simulink model "OL_MMC_dqn_GIThub"  (R2024a)
settings: Solver=FixedStepDiscrete  StartTime=0.0  StopTime=2.5  RelTol=1e-3
values from neighbouring files (symbols this model uses):
  f1 = fg    [mmc_dp_hss_vs_simulink_dqn.m]
  fg = 50    [OL_TD_DP_HSS_dqn.m]
  fh = 150    [mmc_dp_hss_vs_simulink_dqn.m]
  flag_hAC = 0    [mmc_dp_hss_vs_simulink_dqn.m]
  il0 = zSS0(4:6)    [mmc_dp_hss_vs_simulink_dqn.m]
  iu0 = zSS0(1:3)    [mmc_dp_hss_vs_simulink_dqn.m]
  kdcL = 1    [mmc_dp_hss_vs_simulink_dqn.m]
  Low_arm_gain = Nsm/Csm    [mmc_dp_hss_vs_simulink_dqn.m]
  m = 0.85    [OL_TD_DP_HSS_dqn.m]
  mStepRel = 0    [mmc_dp_hss_vs_simulink_dqn.m]
  N = 1    [mmc_dp_hss_vs_simulink_dqn.m]
  p = [p, i]    [OL_TD_DP_HSS_dqn.m]
  phMod = pi/2 + delta + [0, -2*pi/3, 2*pi/3]    [mmc_dp_hss_vs_simulink_dqn.m]
  SOL =     [SOL.mat]
  su = -1    [mmc_dp_hss_vs_simulink_dqn.m]
  su_f = -1    [mmc_dp_hss_vs_simulink_dqn.m]
  T_dc = 0.66    [mmc_dp_hss_vs_simulink_dqn.m]
  t_entranceHF = 0.65    [mmc_dp_hss_vs_simulink_dqn.m]
  Ts_log = Tp/M    [mmc_dp_hss_vs_simulink_dqn.m]
  tStep = Tss    (= 0.6)    [mmc_dp_hss_vs_simulink_dqn.m]
  vC0_sl = zSS0(7:12)    [mmc_dp_hss_vs_simulink_dqn.m]
  Vg_sim = complex([[0 1i*Vpeak; 0 0; 0 0], zeros(3, N+2)])    [mmc_dp_hss_vs_simulink_dqn.m]
  Vpeak = Vac_pk    [mmc_dp_hss_vs_simulink_dqn.m]
undefined symbols (not defined in the file or in its folder): DiscIntNeverNeededParam, S, SY3
libraries: DQsym_Lib x19, spsControlledVoltageSourceLib x11, spsSeriesRLCBranchLib x10, spsCurrentMeasurementLib x6, spsGroundLib x4, spsThreePhaseVIMeasurementLib x1, spspowerguiLib x1
settings Model: Creator=salsarayreh  LastModifiedBy=salsarayreh
settings DataIOCC: SaveFinalState=on  SaveOperatingPoint=on  SaveFormat=Array  SaveState=on  ReturnWorkspaceOutputs=off

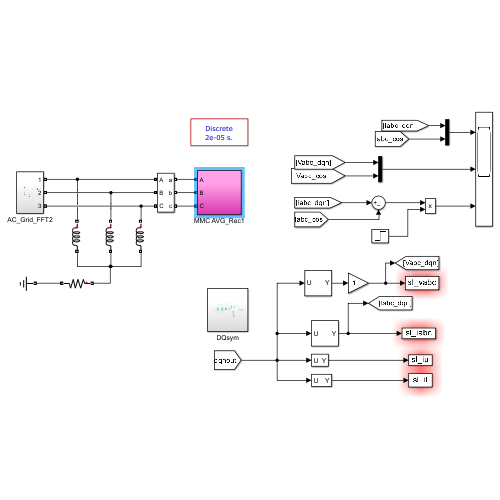
[thumbnail: Simulink's stored preview of the top-level diagram]
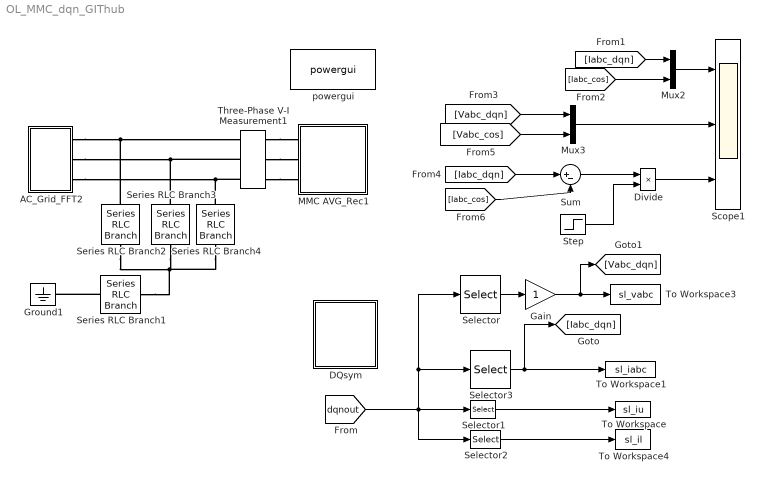
== system OL_MMC_dqn_GIThub ==
  AC_Grid_FFT2 : Subsystem
  DQsym : Subsystem
  Divide : Product  Inputs=**
  Gain : Gain
  Ground1 : spsGroundLib/Ground  LConnTagsString=a
  MMC AVG_Rec1 : Subsystem
  Mux2 : Mux  Inputs=2
  Mux3 : Mux  Inputs=2
  Scope1 : Scope  NumInputPorts=3
  Selector : Selector  InputPortWidth=12  IndexOptions=Index vector (dialog)  Indices=[1:3]  OutputSizes=1
  Selector1 : Selector  InputPortWidth=12  IndexOptions=Index vector (dialog)  Indices=[4:6]  OutputSizes=1
  Selector2 : Selector  InputPortWidth=12  IndexOptions=Index vector (dialog)  Indices=[7:9]  OutputSizes=1
  Selector3 : Selector  InputPortWidth=12  IndexOptions=Index vector (dialog)  Indices=[10:12]  OutputSizes=1
  Series RLC Branch1 : spsSeriesRLCBranchLib/Series RLC Branch  LConnTagsString=__new0  RConnTagsString=__new0  BranchType=R  Resistance=10  Inductance=1e-3  SetiL0=off  InitialCurrent=0  Capacitance=1e-6  Setx0=off  InitialVoltage=0  Measurements=None
  Series RLC Branch2 : spsSeriesRLCBranchLib/Series RLC Branch  LConnTagsString=__new0  RConnTagsString=__new0  BranchType=L  Resistance=10  Inductance=5  SetiL0=off  InitialCurrent=0  Capacitance=1e-6  Setx0=off  InitialVoltage=0  Measurements=None
  Series RLC Branch3 : spsSeriesRLCBranchLib/Series RLC Branch  LConnTagsString=__new0  RConnTagsString=__new0  BranchType=L  Resistance=10  Inductance=5  SetiL0=off  InitialCurrent=0  Capacitance=1e-6  Setx0=off  InitialVoltage=0  Measurements=None
  Series RLC Branch4 : spsSeriesRLCBranchLib/Series RLC Branch  LConnTagsString=__new0  RConnTagsString=__new0  BranchType=L  Resistance=10  Inductance=5  SetiL0=off  InitialCurrent=0  Capacitance=1e-6  Setx0=off  InitialVoltage=0  Measurements=None
  Step : Step  Time=0.5  SampleTime=0
  Sum : Sum  Inputs=|+-
  Three-Phase V-I Measurement1 : spsThreePhaseVIMeasurementLib/Three-Phase V-I Measurement  VoltageMeasurement=phase-to-ground  SetLabelV=on  LabelV=Vabc_cos  Vpu=off  VpuLL=off  CurrentMeasurement=yes  SetLabelI=on  LabelI=Iabc_cos  Ipu=off  Pbase=100e6  Vbase=500e3  OutputType=Complex  PhasorSimulation=off  PSBequivalent=0
  To Workspace : ToWorkspace  VariableName=sl_iu  SaveFormat=Timeseries  SampleTime=Ts_log
  To Workspace1 : ToWorkspace  VariableName=sl_iabc  SaveFormat=Timeseries  SampleTime=Ts_log
  To Workspace3 : ToWorkspace  VariableName=sl_vabc  SaveFormat=Timeseries  SampleTime=Ts_log
  To Workspace4 : ToWorkspace  VariableName=sl_il  SaveFormat=Timeseries  SampleTime=Ts_log
  powergui : spspowerguiLib/powergui  Priority=1  SimulationMode=Discrete  SampleTime=2e-5  frequency=60  Iterations=50  frequencyindice=0  Pbase=100e6  ErrMax=1e-4  UnitsV=kV  UnitsW=MW  buscounter=0  FunctionMessages=off  echomessages=off  EnableUseOfTLC=off  CurrentSourceSwitches=off  DisableSnubberDevices=off  DisableRonSwitches=off  DisableVfSwitches=off  DisplayEquations=off  AutomaticDiscreteSolvers=off  SolverType=Tustin/Backward Euler (TBE)  Interpol=off  ExternalGateDelay=off  methode=off  Ts=10  x0status=blocks  SPID=off  SwTol=0  HookPort=off  NonlinearTolerance=1e-4  nMaxIteration=100  ContinueOnMaxIteration=off  RestoreLinks=warning  ResistiveCurrentMeasurement=off  Frange=[0:2:500]  Ylog=off  Xlog=on  ShowGrid=off  save=off  variable=ZData  structure=VIprim  ZoomFFT=on  StartTime=0.15  cycles=2  DisplayStyle=1  fundamental=50  FreqAxis=on  MaxFrequency=1000  frequencyindicesteady=1  RmsSteady=1  display=off
  wires:
  Selector3/1 -> To Workspace1/1, [Iabc_dqn]
  Selector/1 -> Gain/1
  Gain/1 -> [Vabc_dqn], To Workspace3/1
  [dqnout] -> Selector/1, Selector3/1, Selector2/1, Selector1/1
  [Vabc_cos] -> Mux3/2
  [Iabc_cos] -> Mux2/2
  Mux2/1 -> Scope1/1
  Mux3/1 -> Scope1/2
  Selector2/1 -> To Workspace4/1
  Selector1/1 -> To Workspace/1
  Divide/1 -> Scope1/3
  Sum/1 -> Divide/1
  Step/1 -> Divide/2
  [Iabc_dqn] -> Mux2/1
  [Vabc_dqn] -> Mux3/1
  [Iabc_dqn] -> Sum/1
  [Iabc_cos] -> Sum/2
  connections:
  Series RLC Branch1/LConn1 -- Series RLC Branch2/RConn1 -- Series RLC Branch4/RConn1 -- Series RLC Branch3/RConn1
  Three-Phase V-I Measurement1/LConn2 -- Series RLC Branch3/LConn1 -- AC_Grid_FFT2/LConn2
  Three-Phase V-I Measurement1/LConn3 -- AC_Grid_FFT2/LConn3 -- Series RLC Branch4/LConn1
  AC_Grid_FFT2/LConn1 -- Three-Phase V-I Measurement1/LConn1 -- Series RLC Branch2/LConn1
  Series RLC Branch1/RConn1 -- Ground1/LConn1
  Three-Phase V-I Measurement1/RConn2 -- MMC AVG_Rec1/LConn2
  Three-Phase V-I Measurement1/RConn3 -- MMC AVG_Rec1/LConn3
  Three-Phase V-I Measurement1/RConn1 -- MMC AVG_Rec1/LConn1

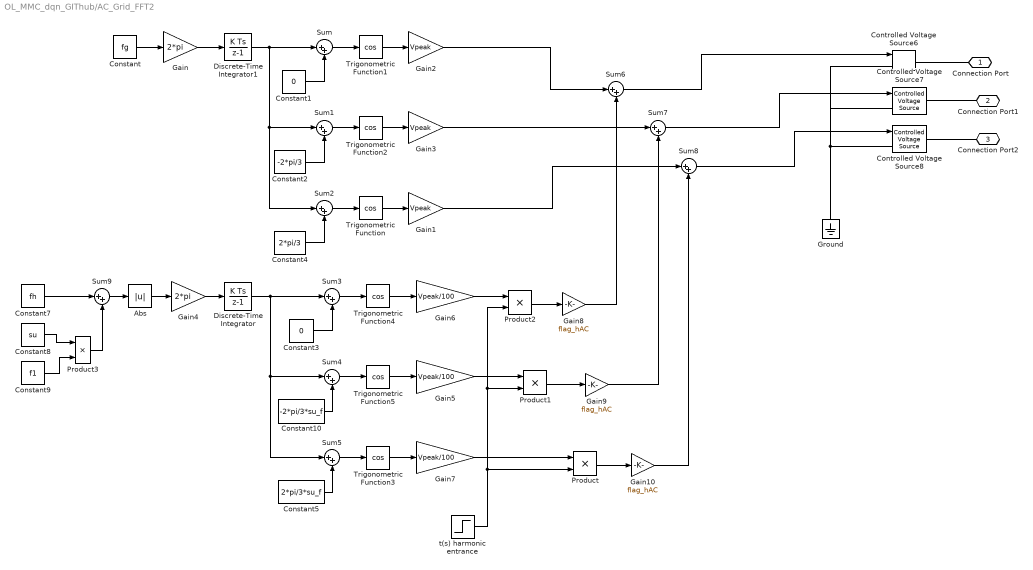
== system OL_MMC_dqn_GIThub/AC_Grid_FFT2 ==
  Abs : Abs  SaturateOnIntegerOverflow=off
  Constant : Constant  Value=fg
  Constant1 : Constant  Value=0
  Constant10 : Constant  Value=-2*pi/3*su_f
  Constant2 : Constant  Value=-2*pi/3
  Constant3 : Constant  Value=0
  Constant4 : Constant  Value=2*pi/3
  Constant5 : Constant  Value=2*pi/3*su_f
  Constant7 : Constant  Value=fh
  Constant8 : Constant  Value=su
  Constant9 : Constant  Value=f1
  Controlled Voltage Source6 : spsControlledVoltageSourceLib/Controlled Voltage Source  Initialize=on  Source_Type=AC  Amplitude=0  Phase=0  Frequency=0  Measurements=None
  Controlled Voltage Source7 : spsControlledVoltageSourceLib/Controlled Voltage Source  Initialize=on  Source_Type=AC  Amplitude=0  Phase=0  Frequency=0  Measurements=None
  Controlled Voltage Source8 : spsControlledVoltageSourceLib/Controlled Voltage Source  Initialize=on  Source_Type=AC  Amplitude=0  Phase=0  Frequency=0  Measurements=None
  Discrete-Time Integrator : DiscreteIntegrator  SampleTime=-1  ICPrevOutput=DiscIntNeverNeededParam  ICPrevScaledInput=DiscIntNeverNeededParam
  Discrete-Time Integrator1 : DiscreteIntegrator  SampleTime=-1  ICPrevOutput=DiscIntNeverNeededParam  ICPrevScaledInput=DiscIntNeverNeededParam
  Gain : Gain  Gain=2*pi
  Gain1 : Gain  Gain=Vpeak
  Gain10 : Gain  Gain=flag_hAC
  Gain2 : Gain  Gain=Vpeak
  Gain3 : Gain  Gain=Vpeak
  Gain4 : Gain  Gain=2*pi
  Gain5 : Gain  Gain=Vpeak/100
  Gain6 : Gain  Gain=Vpeak/100
  Gain7 : Gain  Gain=Vpeak/100
  Gain8 : Gain  Gain=flag_hAC
  Gain9 : Gain  Gain=flag_hAC
  Ground : spsGroundLib/Ground  LConnTagsString=a
  Product{,1..3} (4 alike) : Product
  Sum{,1..9} (10 alike) : Sum  Inputs=|++
  Trigonometric Function{,1..5} (6 alike) : Trigonometry  Operator=cos
  t(s) harmonic entrance : Step  Time=t_entranceHF  SampleTime=0
  Connection Port : PMIOPort  Side=Left
  Connection Port1 : PMIOPort  Port=2  Side=Left
  Connection Port2 : PMIOPort  Port=3  Side=Left
  wires:
  Constant9/1 -> Product3/2
  Product3/1 -> Sum9/2
  Constant8/1 -> Product3/1
  Sum9/1 -> Abs/1
  Constant7/1 -> Sum9/1
  Abs/1 -> Gain4/1
  t(s) harmonic entrance/1 -> Product1/2, Product2/2, Product/2
  Gain5/1 -> Product1/1
  Gain6/1 -> Product2/1
  Constant5/1 -> Sum5/2
  Trigonometric Function1/1 -> Gain2/1
  Constant3/1 -> Sum3/2
  Sum4/1 -> Trigonometric Function5/1
  Discrete-Time Integrator1/1 -> Sum/1, Sum1/1, Sum2/1
  Constant2/1 -> Sum1/2
  Constant10/1 -> Sum4/2
  Constant4/1 -> Sum2/2
  Sum2/1 -> Trigonometric Function/1
  Trigonometric Function3/1 -> Gain7/1
  Sum/1 -> Trigonometric Function1/1
  Trigonometric Function2/1 -> Gain3/1
  Gain/1 -> Discrete-Time Integrator1/1
  Sum5/1 -> Trigonometric Function3/1
  Constant/1 -> Gain/1
  Trigonometric Function/1 -> Gain1/1
  Sum3/1 -> Trigonometric Function4/1
  Gain4/1 -> Discrete-Time Integrator/1
  Gain3/1 -> Sum7/1
  Gain2/1 -> Sum6/1
  Trigonometric Function5/1 -> Gain5/1
  Trigonometric Function4/1 -> Gain6/1
  Constant1/1 -> Sum/2
  Gain7/1 -> Product/1
  Gain1/1 -> Sum8/1
  Sum1/1 -> Trigonometric Function2/1
  Discrete-Time Integrator/1 -> Sum5/1, Sum4/1, Sum3/1
  Product2/1 -> Gain8/1
  Product1/1 -> Gain9/1
  Product/1 -> Gain10/1
  Sum6/1 -> Controlled Voltage Source6/1
  Sum8/1 -> Controlled Voltage Source8/1
  Sum7/1 -> Controlled Voltage Source7/1
  Gain8/1 -> Sum6/2
  Gain9/1 -> Sum7/2
  Gain10/1 -> Sum8/2
  connections:
  Ground/LConn1 -- Controlled Voltage Source6/LConn1 -- Controlled Voltage Source7/LConn1 -- Controlled Voltage Source8/LConn1
  Connection Port/RConn1 -- Controlled Voltage Source6/RConn1
  Connection Port1/RConn1 -- Controlled Voltage Source7/RConn1
  Connection Port2/RConn1 -- Controlled Voltage Source8/RConn1

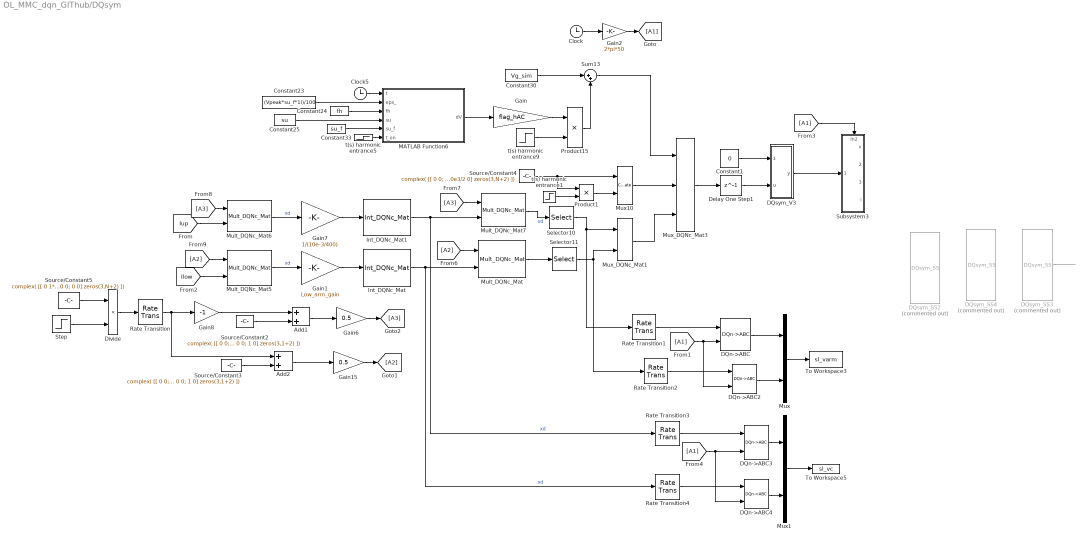
== system OL_MMC_dqn_GIThub/DQsym ==
  Add1 : Sum
  Add2 : Sum
  Clock : Clock
  Clock5 : Clock
  Constant1 : Constant  Value=0
  Constant23 : Constant  Value=(Vpeak*su_f*1i)/100
  Constant24 : Constant  Value=fh
  Constant25 : Constant  Value=su
  Constant30 : Constant  Value=Vg_sim
  Constant33 : Constant  Value=su_f
  DQn->ABC{,2..4} (4 alike) : DQsym_Lib/DQn->ABC  N=4
      settings: SourceProductName=DQsym Library
  DQsym_SS2 : DQsym_Lib/DQsym_SS  Commented=on  Ad=SOL.A  Bd=SOL.B  Cd=SOL.C  Dd=SOL.D  f=fg  swOnRes=0  swOffRes=0  swType=0  Ts=2e-5  nrSWvec=0  xo=SOL.x0
      settings: SourceProductName=DQsym Library
  DQsym_SS3 : DQsym_Lib/DQsym_SS  Commented=on  Ad=Ad1  Bd=Bd1  Cd=Cd1  Dd=Dd1  f=Fnom  swOnRes=1e-3*ones(1,6)  swOffRes=1e6*ones(1,6)  swType=zeros(1,6)  Ts=2e-5  nrSWvec=0  xo=zeros(6,1)
      settings: SourceProductName=DQsym Library
  DQsym_SS4 : DQsym_Lib/DQsym_SS  Commented=on  Ad=ds.A  Bd=ds.B  Cd=ds.C  Dd=ds.D  f=Fnom  swOnRes=1e-3*ones(1,6)  swOffRes=1e6*ones(1,6)  swType=zeros(1,6)  Ts=2e-5  nrSWvec=0  xo=zeros(6,1)
      settings: SourceProductName=DQsym Library
  DQsym_V3 : MATLAB Function  AncestorBlock=DQsym_Lib/DQsym_V3  TreatAsAtomicUnit=on  mask{Ad=SOL.A, Bd=SOL.B, Cd=SOL.C, Dd=SOL.D, f=50, swOnRes=0, swOffRes=0, swType=0, Ts=2e-5, nrSWvec=0, xo=zeros(9,1)}
      mask prompts: Ad "A"; Bd "B"; Cd "C"; Dd "D"; f "frequency"; swOnRes "Switch on resistance:"; swOffRes "Switch off resistance:"; swType "Switch type:"; Ts "Time step (s):"; nrSWvec "Number of switches:"; xo "Initial conditions"
  Delay One Step1 : Delay  DelayLength=1  SampleTime=2e-5
  Divide : Product  Inputs=**
  Gain : Gain  Gain=flag_hAC
  Gain1 : Gain  Gain=Low_arm_gain
  Gain15 : Gain  Gain=0.5
  Gain2 : Gain  Gain=2*pi*50
  Gain6 : Gain  Gain=0.5
  Gain7 : Gain  Gain=1/(10e-3/400)
  Gain8 : Gain  Gain=-1
  Int_DQNc_Mat : DQsym_Lib/Int_DQNc_Mat  N=N+7  dt=Ts_dqn  w=2*pi*fg  InitInt=[vC0_sl(4) ;vC0_sl(5);vC0_sl(6)]  swFeed=off  R=eye(3)  iL=eye(3)
      settings: SourceProductName=DQsym Library
  Int_DQNc_Mat1 : DQsym_Lib/Int_DQNc_Mat  N=N+7  dt=Ts_dqn  w=2*pi*fg  InitInt=[vC0_sl(1) ;vC0_sl(2);vC0_sl(3)]  swFeed=off  R=eye(3)  iL=eye(3)
      settings: SourceProductName=DQsym Library
  MATLAB Function6 : MATLAB Function  TreatAsAtomicUnit=on
  Mult_DQNc_Mat : DQsym_Lib/Mult_DQNc_Mat  N=N+9  HrmDbl=on
      settings: SourceProductName=DQsym Library
  Mult_DQNc_Mat5 : DQsym_Lib/Mult_DQNc_Mat  N=N+3  HrmDbl=on
      settings: SourceProductName=DQsym Library
  Mult_DQNc_Mat6 : DQsym_Lib/Mult_DQNc_Mat  N=N+3  HrmDbl=on
      settings: SourceProductName=DQsym Library
  Mult_DQNc_Mat7 : DQsym_Lib/Mult_DQNc_Mat  N=N+9  HrmDbl=on
      settings: SourceProductName=DQsym Library
  Mux : Mux  Inputs=2
  Mux1 : Mux  Inputs=2
  Mux10 : Concatenate  Mode=Multidimensional array
  Mux_DQNc_Mat1 : DQsym_Lib/Mux_DQNc_Mat  nrInp=2
      settings: SourceProductName=DQsym Library
  Mux_DQNc_Mat3 : DQsym_Lib/Mux_DQNc_Mat  nrInp=3
      settings: SourceProductName=DQsym Library
  Product1 : Product
  Product15 : Product
  Rate Transition : RateTransition  OutPortSampleTime=4e-5
  Rate Transition{1..4} (4 alike) : RateTransition  OutPortSampleTime=2e-5
  Selector10 : Selector  NumberOfDimensions=2  InputPortWidth=size(SY3.C,1)  IndexOptions=Select all,Index vector (dialog)  Indices=4:6,1:N+4  OutputSizes=1,1
  Selector11 : Selector  NumberOfDimensions=2  InputPortWidth=size(SY3.C,1)  IndexOptions=Select all,Index vector (dialog)  Indices=4:6,1:N+4  OutputSizes=1,1
  Source/Constant2 : Constant  Value=complex( [[ 0 0; 0 0; 1 0] zeros(3,1+2) ])
  Source/Constant3 : Constant  Value=complex( [[ 0 0; 0 0; 1 0] zeros(3,1+2) ])
  Source/Constant4 : Constant  Value=complex( [[ 0 0; 0 0; 640e3/2 0] zeros(3,N+2) ])
  Source/Constant5 : Constant  Value=complex( [[ 0 1*exp(1i*1.5359); 0 0; 0 0] zeros(3,N+2) ])
  Step : Step  Time=tStep  Before=m  After=m*(1+mStepRel)  SampleTime=0
  Subsystem3 : Subsystem
      settings: PortSchema="{\"entries\":[{\"content\":{\"sides\":[{\"content\":{\"connectorIds\":[\"In1\"]},\"type\":\"ConnectorPlacement.EquallySpacedRectSide\",\"uuid\":\"3bb77d8f-1aaa-4265-9b68-ea1550baad0f\"},{\"content\":{\"connectorIds\":[\"Out1\",\"Out2\",\"Out3\",\"Out4\"],\"side\":\"RIGHT\"},\"type\":\"ConnectorPlacement.EquallySpacedRectSide\",\"uuid\":\"cf9e0e6c-58d6-47ae-94f0-731f989c2c33\"},{\"content\":{\"connectorIds\":[\"In2\"],\"side\":\"TOP\"},\"type\":\"ConnectorPlacement.EquallySpacedRectSide\",\"uuid\":\"a148aa31-b036-466e-b1e9-6b0bda301938\"}]},\"type\":\"ConnectorPlacement.EquallySpacedConnector\",\"uuid\":\"1e5021a9-33df-40ee-a00e-8c2f12721673\"}],\"packageUris\":[\"http://schema.mathworks.com/mf0/Connector/R2020b\"],\"version\":\"1.0\"}"
  Sum13 : Sum  Inputs=|++
  To Workspace3 : ToWorkspace  VariableName=sl_varm  SaveFormat=Timeseries  SampleTime=Ts_log
  To Workspace5 : ToWorkspace  VariableName=sl_vc  SaveFormat=Timeseries  SampleTime=Ts_log
  t(s) harmonic entrance1 : Step  Time=T_dc  Before=1  After=kdcL  SampleTime=0
  t(s) harmonic entrance5 : Step  Time=t_entranceHF  SampleTime=0
  t(s) harmonic entrance9 : Step  Time=t_entranceHF  SampleTime=0
  wires:
  Int_DQNc_Mat1/1 -> Mult_DQNc_Mat7/2, Rate Transition3/1  "xd"
  [A3] -> Mult_DQNc_Mat7/1
  Int_DQNc_Mat/1 -> Mult_DQNc_Mat/2, Rate Transition4/1  "xd"
  Mult_DQNc_Mat5/1 -> Gain1/1  "xd"
  Constant1/1 -> DQsym_V3/1(brkVec)
  [A3] -> Mult_DQNc_Mat6/1
  [Ilow] -> Mult_DQNc_Mat5/2
  Delay One Step1/1 -> DQsym_V3/2(u)
  Selector10/1 -> Mux_DQNc_Mat1/1, Rate Transition1/1
  DQsym_SS3/1 -> ?
  [A2] -> Mult_DQNc_Mat5/1
  [A2] -> Mult_DQNc_Mat/1
  [A1] -> Subsystem3/2(In2)
  Mult_DQNc_Mat7/1 -> Selector10/1  "xd"
  Sum13/1 -> Mux_DQNc_Mat3/1
  ? -> DQsym_SS3/1
  Gain7/1 -> Int_DQNc_Mat1/1
  Selector11/1 -> Mux_DQNc_Mat1/2, Rate Transition2/1
  ? -> DQsym_SS3/2
  Mux_DQNc_Mat3/1 -> Delay One Step1/1
  [Iup] -> Mult_DQNc_Mat6/2
  DQsym_V3/1(y) -> Subsystem3/1(In1)
  Mult_DQNc_Mat6/1 -> Gain7/1  "xd"
  Gain1/1 -> Int_DQNc_Mat/1
  Mult_DQNc_Mat/1 -> Selector11/1
  Mux_DQNc_Mat1/1 -> Mux_DQNc_Mat3/3
  Gain2/1 -> [A1]
  [A1] -> DQn->ABC2/2, DQn->ABC/2
  Clock/1 -> Gain2/1
  Add1/1 -> Gain6/1
  Gain15/1 -> [A2]
  Gain6/1 -> [A3]
  Divide/1 -> Rate Transition/1
  Add2/1 -> Gain15/1
  Source/Constant3/1 -> Add2/2
  Gain8/1 -> Add1/1
  Source/Constant2/1 -> Add1/2
  Step/1 -> Divide/2
  Source/Constant5/1 -> Divide/1
  Mux10/1 -> Mux_DQNc_Mat3/2
  Source/Constant4/1 -> Mux10/1, Product1/1
  DQn->ABC/1 -> Mux/1
  DQn->ABC2/1 -> Mux/2
  Mux/1 -> To Workspace3/1
  Rate Transition/1 -> Add2/1, Gain8/1
  Rate Transition1/1 -> DQn->ABC/1
  Rate Transition2/1 -> DQn->ABC2/1
  Rate Transition4/1 -> DQn->ABC4/1
  Rate Transition3/1 -> DQn->ABC3/1
  Mux1/1 -> To Workspace5/1
  DQn->ABC4/1 -> Mux1/2
  DQn->ABC3/1 -> Mux1/1
  [A1] -> DQn->ABC3/2, DQn->ABC4/2
  Clock5/1 -> MATLAB Function6/1(t)
  Constant33/1 -> MATLAB Function6/5(su_f)
  t(s) harmonic entrance5/1 -> MATLAB Function6/6(t_on)
  Constant23/1 -> MATLAB Function6/2(eps_)
  Constant25/1 -> MATLAB Function6/4(su)
  t(s) harmonic entrance9/1 -> Product15/2
  Constant24/1 -> MATLAB Function6/3(fh)
  Product15/1 -> Sum13/2
  MATLAB Function6/1(dV) -> Gain/1
  Constant30/1 -> Sum13/1
  Gain/1 -> Product15/1
  t(s) harmonic entrance1/1 -> Product1/2
  Product1/1 -> Mux10/2

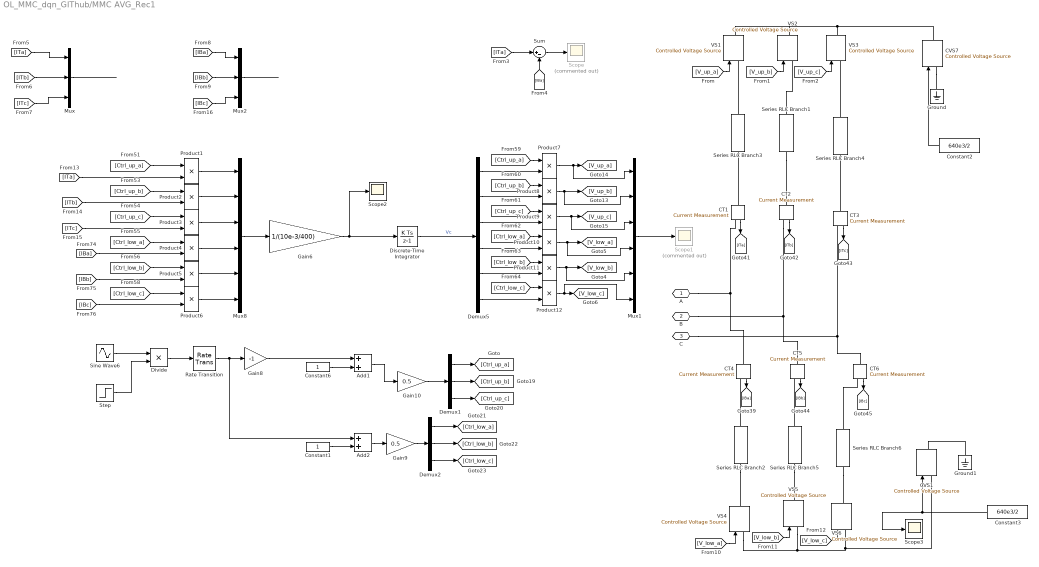
== system OL_MMC_dqn_GIThub/MMC AVG_Rec1 ==
  Add1 : Sum
  Add2 : Sum
  CT{1..6} (6 alike) : spsCurrentMeasurementLib/Current Measurement  PhasorSimulation=off  OutputType=Complex  PSBequivalent=0
  CVS1 : spsControlledVoltageSourceLib/Controlled Voltage Source  Initialize=off  Source_Type=AC  Amplitude=0  Phase=0  Frequency=0  Measurements=None
  CVS7 : spsControlledVoltageSourceLib/Controlled Voltage Source  Initialize=off  Source_Type=AC  Amplitude=0  Phase=0  Frequency=0  Measurements=None
  Constant1 : Constant
  Constant2 : Constant  Value=640e3/2  SampleTime=2e-5
  Constant3 : Constant  Value=640e3/2  SampleTime=2e-5
  Constant6 : Constant
  Demux1 : Demux  Outputs=3
  Demux2 : Demux  Outputs=3
  Demux5 : Demux  Outputs=6
  Discrete-Time Integrator : DiscreteIntegrator  InitialCondition=vC0_sl  SampleTime=-1  ICPrevOutput=DiscIntNeverNeededParam  ICPrevScaledInput=DiscIntNeverNeededParam
  Divide : Product  Inputs=**
  Gain10 : Gain  Gain=0.5
  Gain6 : Gain  Gain=1/(10e-3/400)
  Gain8 : Gain  Gain=-1
  Gain9 : Gain  Gain=0.5
  Ground : spsGroundLib/Ground  LConnTagsString=a
  Ground1 : spsGroundLib/Ground  LConnTagsString=a
  Mux : Mux  Inputs=3
  Mux1 : Mux  Inputs=6
  Mux2 : Mux  Inputs=3
  Mux8 : Mux  Inputs=6
  Product{1..12} (12 alike) : Product
  Rate Transition : RateTransition  OutPortSampleTime=4e-5
  Scope : Scope  Commented=on
  Scope1 : Scope  Commented=on
  Scope2 : Scope
  Scope3 : Scope
  Series RLC Branch1 : spsSeriesRLCBranchLib/Series RLC Branch  LConnTagsString=__new0  RConnTagsString=__new0  BranchType=RL  Resistance=1.07  Inductance=50e-3  SetiL0=on  InitialCurrent=iu0(p)  Capacitance=1e-6  Setx0=off  InitialVoltage=0  Measurements=None
  Series RLC Branch2 : spsSeriesRLCBranchLib/Series RLC Branch  LConnTagsString=__new0  RConnTagsString=__new0  BranchType=RL  Resistance=1.07  Inductance=50e-3  SetiL0=on  InitialCurrent=il0(p)  Capacitance=1e-6  Setx0=off  InitialVoltage=0  Measurements=None
  Series RLC Branch3 : spsSeriesRLCBranchLib/Series RLC Branch  LConnTagsString=__new0  RConnTagsString=__new0  BranchType=RL  Resistance=1.07  Inductance=50e-3  SetiL0=on  InitialCurrent=iu0(p)  Capacitance=1e-6  Setx0=off  InitialVoltage=0  Measurements=None
  Series RLC Branch4 : spsSeriesRLCBranchLib/Series RLC Branch  LConnTagsString=__new0  RConnTagsString=__new0  BranchType=RL  Resistance=1.07  Inductance=50e-3  SetiL0=on  InitialCurrent=iu0(p)  Capacitance=1e-6  Setx0=off  InitialVoltage=0  Measurements=None
  Series RLC Branch5 : spsSeriesRLCBranchLib/Series RLC Branch  LConnTagsString=__new0  RConnTagsString=__new0  BranchType=RL  Resistance=1.07  Inductance=50e-3  SetiL0=on  InitialCurrent=il0(p)  Capacitance=1e-6  Setx0=off  InitialVoltage=0  Measurements=None
  Series RLC Branch6 : spsSeriesRLCBranchLib/Series RLC Branch  LConnTagsString=__new0  RConnTagsString=__new0  BranchType=RL  Resistance=1.07  Inductance=50e-3  SetiL0=on  InitialCurrent=il0(p)  Capacitance=1e-6  Setx0=off  InitialVoltage=0  Measurements=None
  Sine Wave6 : Sin  Amplitude=1 *ones(1,3)  Frequency=2*pi*50  Phase=phMod  SampleTime=0
  Step : Step  Time=tStep  Before=m  After=m*(1+mStepRel)  SampleTime=0
  Sum : Sum  Inputs=|+-
  VS{1..6} (6 alike) : spsControlledVoltageSourceLib/Controlled Voltage Source  Initialize=on  Source_Type=AC  Amplitude=0  Phase=0  Frequency=0  Measurements=None
  A : PMIOPort  Side=Left
  B : PMIOPort  Port=2  Side=Left
  C : PMIOPort  Port=3  Side=Left
  wires:
  CT6/1 -> [IBc]
  CT5/1 -> [IBb]
  CT3/1 -> [ITc]
  CT2/1 -> [ITb]
  CT1/1 -> [ITa]
  CT4/1 -> [IBa]
  Product12/1 -> Mux1/6, [V_low_c]
  Demux5/5 -> Product11/2
  Product8/1 -> Mux1/2, [V_up_b]
  [Ctrl_low_b] -> Product5/1
  Product3/1 -> Mux8/3
  [Ctrl_low_a] -> Product10/1
  [Ctrl_up_b] -> Product8/1
  Demux5/6 -> Product12/2
  Demux5/3 -> Product9/2
  [Ctrl_up_a] -> Product7/1
  Product11/1 -> Mux1/5, [V_low_b]
  [Ctrl_up_c] -> Product9/1
  Product6/1 -> Mux8/6
  Product2/1 -> Mux8/2
  [Ctrl_up_c] -> Product3/1
  [Ctrl_low_a] -> Product4/1
  [Ctrl_up_b] -> Product2/1
  [Ctrl_low_c] -> Product6/1
  [Ctrl_up_a] -> Product1/1
  Product10/1 -> Mux1/4, [V_low_a]
  Discrete-Time Integrator/1 -> Demux5/1  "Vc"
  Demux5/4 -> Product10/2
  Product4/1 -> Mux8/4
  Product5/1 -> Mux8/5
  Mux8/1 -> Gain6/1
  Product9/1 -> Mux1/3, [V_up_c]
  Demux5/2 -> Product8/2
  [Ctrl_low_c] -> Product12/1
  Product1/1 -> Mux8/1
  [Ctrl_low_b] -> Product11/1
  Product7/1 -> Mux1/1, [V_up_a]
  Demux5/1 -> Product7/2
  Gain6/1 -> Discrete-Time Integrator/1, Scope2/1
  [V_low_c] -> VS6/1
  [V_up_b] -> VS2/1
  [V_low_b] -> VS5/1
  [V_up_a] -> VS1/1
  [V_low_a] -> VS4/1
  [V_up_c] -> VS3/1
  Add1/1 -> Gain10/1
  Demux2/3 -> [Ctrl_low_c]
  Demux1/1 -> [Ctrl_up_a]
  Add2/1 -> Gain9/1
  Demux1/3 -> [Ctrl_up_c]
  Demux2/1 -> [Ctrl_low_a]
  Gain9/1 -> Demux2/1
  Demux1/2 -> [Ctrl_up_b]
  Constant1/1 -> Add2/2
  Demux2/2 -> [Ctrl_low_b]
  Constant6/1 -> Add1/2
  Gain8/1 -> Add1/1
  Gain10/1 -> Demux1/1
  [IBc] -> Product6/2
  [IBb] -> Product5/2
  [IBa] -> Product4/2
  [ITc] -> Product3/2
  [ITb] -> Product2/2
  [ITa] -> Product1/2
  [IBa] -> Sum/2
  [ITa] -> Sum/1
  Sum/1 -> Scope/1
  Mux1/1 -> Scope1/1
  Divide/1 -> Rate Transition/1
  [ITb] -> Mux/2
  [ITa] -> Mux/1
  [ITc] -> Mux/3
  [IBb] -> Mux2/2
  [IBa] -> Mux2/1
  [IBc] -> Mux2/3
  Sine Wave6/1 -> Divide/1
  Step/1 -> Divide/2
  Rate Transition/1 -> Add2/1, Gain8/1
  Mux/1 -> ?
  Mux2/1 -> ?
  Constant2/1 -> CVS7/1
  Constant3/1 -> Scope3/1, CVS1/1
  connections:
  C/RConn1 -- CT3/RConn1 -- CT6/LConn1
  B/RConn1 -- CT5/LConn1 -- CT2/RConn1
  A/RConn1 -- CT4/LConn1 -- CT1/RConn1
  Series RLC Branch4/LConn1 -- VS3/LConn1
  Series RLC Branch1/LConn1 -- VS2/LConn1
  Series RLC Branch3/LConn1 -- VS1/LConn1
  Series RLC Branch5/RConn1 -- VS5/RConn1
  Series RLC Branch6/RConn1 -- VS6/RConn1
  Series RLC Branch2/RConn1 -- VS4/RConn1
  Series RLC Branch5/LConn1 -- CT5/RConn1
  Series RLC Branch2/LConn1 -- CT4/RConn1
  Series RLC Branch6/LConn1 -- CT6/RConn1
  CVS7/RConn1 -- VS1/RConn1 -- VS2/RConn1 -- VS3/RConn1
  VS5/LConn1 -- CVS1/LConn1 -- VS6/LConn1 -- VS4/LConn1
  CVS7/LConn1 -- Ground/LConn1
  Ground1/LConn1 -- CVS1/RConn1
  CT1/LConn1 -- Series RLC Branch3/RConn1
  CT3/LConn1 -- Series RLC Branch4/RConn1
  Series RLC Branch1/RConn1 -- CT2/LConn1

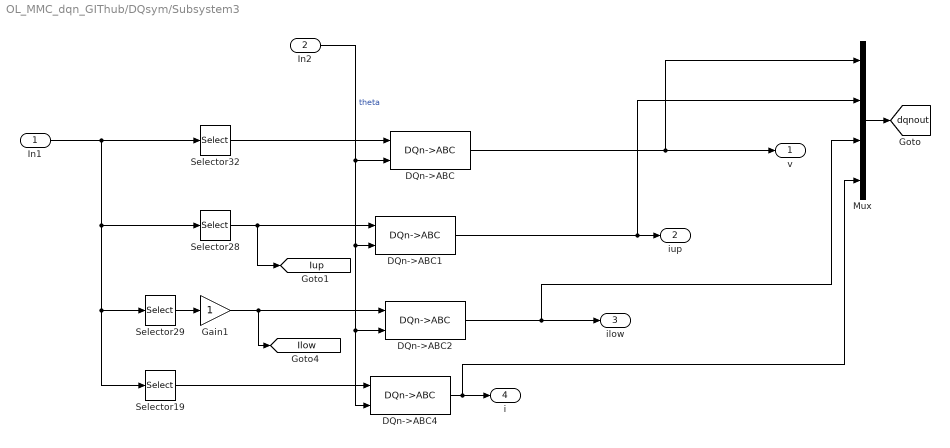
== system OL_MMC_dqn_GIThub/DQsym/Subsystem3 ==
  In1 : Inport
  In2 : Inport  Port=2
  DQn->ABC{,1..2,4} (4 alike) : DQsym_Lib/DQn->ABC  N=N+3
      settings: SourceProductName=DQsym Library
  Gain1 : Gain
  Mux : Mux
  Selector19 : Selector  NumberOfDimensions=2  InputPortWidth=size(S.C,1)  IndexOptions=Index vector (dialog),Select all  Indices=[10:12],1  OutputSizes=1,1
  Selector28 : Selector  NumberOfDimensions=2  InputPortWidth=size(S.C,1)  IndexOptions=Index vector (dialog),Select all  Indices=[4:6],1  OutputSizes=1,1
  Selector29 : Selector  NumberOfDimensions=2  InputPortWidth=size(S.C,1)  IndexOptions=Index vector (dialog),Select all  Indices=[7:9],1  OutputSizes=1,1
  Selector32 : Selector  NumberOfDimensions=2  InputPortWidth=size(S.C,1)  IndexOptions=Index vector (dialog),Select all  Indices=[1:3],1  OutputSizes=1,1
  v : Outport
  iup : Outport  Port=2
  ilow : Outport  Port=3
  i : Outport  Port=4
  tag scope: Ilow=global, Iup=global, dqnout=global
  wires:
  Selector32/1 -> DQn->ABC/1
  In1/1 -> Selector32/1, Selector19/1, Selector29/1, Selector28/1
  In2/1 -> DQn->ABC4/2, DQn->ABC2/2, DQn->ABC1/2, DQn->ABC/2  "theta"
  Selector29/1 -> Gain1/1
  DQn->ABC4/1 -> Mux/4, i/1
  DQn->ABC2/1 -> Mux/3, ilow/1
  Selector19/1 -> DQn->ABC4/1
  Gain1/1 -> [Ilow], DQn->ABC2/1
  Selector28/1 -> [Iup], DQn->ABC1/1
  DQn->ABC/1 -> Mux/1, v/1
  DQn->ABC1/1 -> Mux/2, iup/1
  Mux/1 -> [dqnout]

== matlab function OL_MMC_dqn_GIThub/DQsym/DQsym_V3 ==
  data: Ad parameter; Bd parameter; Cd parameter; Dd parameter; swOnRes parameter; swOffRes parameter; swType parameter; brkVec input; u input; y output [1..100]; xo parameter; f parameter; Ts parameter
function y = nFdss2(Ad, Bd, Cd, Dd, swOnRes, swOffRes, swType, brkVec, u, xo, f, Ts) %#ok<INUSL>

% Persistent storage
persistent A0 B0 C0 D0;        % Original (all switches open) phasor matrices
persistent Ads Bds Cds Dds;    % Active matrices for current switch state
persistent x_old;
persistent swVecOld;
persistent nSwitches;

% -------------------------------------------------------------------------
% INITIALIZATION (first call)
% -------------------------------------------------------------------------
if isempty(x_old)
    % Phasor conversion only once: this is the "default" model
    [A0, B0, C0, D0] = convertToPhasor(Ad, Bd, Cd, Dd, Ts);

    nSwitches = sum(swType == 1);
    x_old     = complex([zeros(size(xo,1),1), xo, zeros(size(xo,1), size(u,2)-2)]);

    % Build active matrices from the originals for the initial switch state
    % (switches that start closed are now correctly applied)
    [Ads, Bds, Cds, Dds] = applySwitches(A0, B0, C0, D0, brkVec, swOnRes, nSwitches);
    swVecOld = brkVec;
end

swVec = brkVec;

% -------------------------------------------------------------------------
% SWITCH EVENT: rebuild matrices from the ORIGINALS (not incrementally)
% -------------------------------------------------------------------------
if nSwitches > 0 && any(swVec ~= swVecOld)

    % First half-step: t - Ts/2, with pre-switching matrices
    xkm12 = halfStep(Ads, Bds, x_old(:,1), u(:,1));

    % Rebuild from defaults -> all-zero swVec returns exactly A0..D0
    [Ads, Bds, Cds, Dds] = applySwitches(A0, B0, C0, D0, swVec, swOnRes, nSwitches);

    % Second half-step: t + Ts/2, with post-switching matrices
    xkp12 = halfStep(Ads, Bds, x_old(:,1), u(:,1));

    x_old(:,1) = 0.5 * (xkm12 + xkp12);
    swVecOld   = swVec;
end

% -------------------------------------------------------------------------
% STATE AND OUTPUT CALCULATION
% -------------------------------------------------------------------------
x  = Ads * x_old + Bds * u;
x2 = x * diag(exp(-1i * 2*pi*f*Ts * (0:size(u,2)-1)));
x_old = x2;

y = Cds * x2 + Dds * u;

end


% =========================================================================
function [A, B, C, D] = applySwitches(A, B, C, D, swVec, swOnRes, nSwitches)
% Apply the closing (conductance feedback) update for every switch that is
% currently ON, starting from the original matrices passed in.
% Switches that are OFF leave the original model untouched.

    for nSw = 1:nSwitches
        if swVec(nSw) == 1
            ysw  = complex(1 / swOnRes(nSw));
            temp = 1 / (1 - D(nSw,nSw) * ysw);

            % Column updates (computed before row nSw is zeroed)
            DxCol      = D(:, nSw) * (ysw * temp);
            DxCol(nSw) = temp;
            BDcol      = B(:, nSw) * ysw;

            % Save and zero row nSw of C and D
            cRow = C(nSw, :);
            dRow = D(nSw, :);
            C(nSw, :) = 0;
            D(nSw, :) = 0;

            % Update C and D
            C = C + DxCol * cRow;
            D = D + DxCol * dRow;

            % Update A and B using the updated row nSw
            A = A + BDcol * C(nSw, :);
            B = B + BDcol * D(nSw, :);
        end
    end
end


% =========================================================================
function xh = halfStep(A, B, x, u)
% 0.5 * ((A + I) * x + B * u)
    xh = 0.5 * ((A + eye(size(A,1))) * x + B * u);
end


% =========================================================================
function [Adc1, Bdc1, Cdc1, Ddc1] = convertToPhasor(A, B, C, D, dt) %#ok<INUSD>

    % Tustin discretization kept for future development
    % I   = eye(size(A, 1));
    % Ad1 = (I - dt*A/2) \ (I + dt*A/2);
    % Bd1 = (I - dt*A/2) \ B * sqrt(dt);
    % Cd1 = sqrt(dt) * C / (I - dt*A/2);
    % Dd1 = D + C / (I - dt*A/2) * (B*dt/2);

    Ad2 = A; Bd2 = B; Cd2 = C; Dd2 = D;   % temp: testing without TBE discretization

    % Convert to DQN / symmetrical components
    a   = -0.5 + 0.866i;
    a2  = -0.5 - 0.866i;
    Sas = [1, a, a2; 1, a2, a; 1, 1, 1] / 3;

    Adc1 = transformMatrix(Ad2, Sas);
    Bdc1 = transformMatrix(Bd2, Sas);
    Cdc1 = transformMatrix(Cd2, Sas);
    Ddc1 = transformMatrix(Dd2, Sas);
end


% =========================================================================
function Mdc = transformMatrix(Md1, Sas)
    rows = size(Md1,1) / 3;
    cols = size(Md1,2) / 3;
    Mdc  = complex(zeros(3*rows, 3*cols));
    for i = 1:rows
        for j = 1:cols
            r = (1:3) + (i-1)*3;
            c = (1:3) + (j-1)*3;
            Mdc(r, c) = Sas * Md1(r, c) / Sas;
        end
    end
end

== matlab function OL_MMC_dqn_GIThub/DQsym/MATLAB Function6 ==
  data: t input; eps_ input; fh input; su input; su_f input; t_on input; dV output
function dV = ac_perturb_sara(t, eps_, fh, su,su_f, t_on)
dV = complex(zeros(3, 4+1));
if t < t_on, return; end
dV(1, 2) = su_f* eps_*exp(1j*su*2*pi*fh*(t - t_on));   % p row, fundamental column
end
